simulink model "pendulum_openloop"  (R2026a)
settings: Solver=VariableStepAuto
values from neighbouring files (symbols this model uses):
  p = [ ... (first row only)    [init_pendulum.m]
  q0 = [ ... (first row only)    [init_pendulum.m]
  qd0 = [ ... (first row only)    [init_pendulum.m]
  u0 = [ ... (first row only)    [init_pendulum.m]
settings Model: Creator=vb  LastModifiedBy=vb

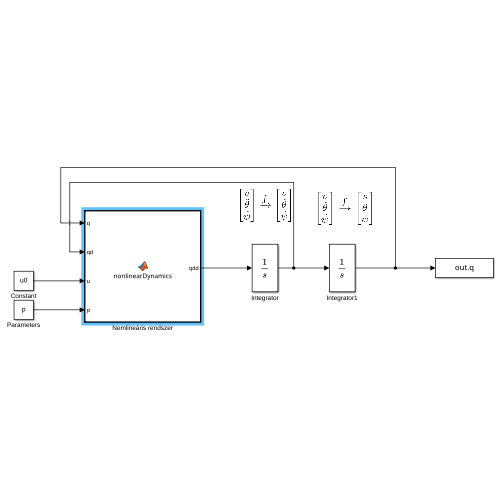
[thumbnail: Simulink's stored preview of the top-level diagram]
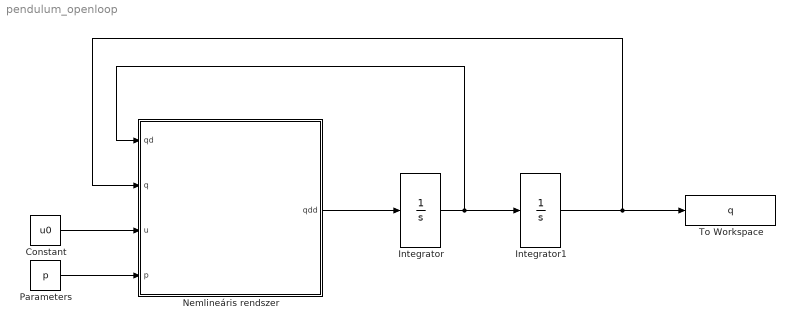
== system pendulum_openloop ==
  Constant : Constant  Value=u0
  Integrator : Integrator  InitialCondition=qd0
  Integrator1 : Integrator  InitialCondition=q0
  Nemlineáris rendszer : MATLAB Function  TreatAsAtomicUnit=on
  Parameters : Constant  Value=p
  To Workspace : ToWorkspace  VariableName=q  SaveFormat=Timeseries  SampleTime=-1
  wires:
  Nemlineáris rendszer/1(qdd) -> Integrator/1
  Integrator/1 -> Nemlineáris rendszer/1(qd), Integrator1/1
  Integrator1/1 -> To Workspace/1, Nemlineáris rendszer/2(q)
  Constant/1 -> Nemlineáris rendszer/3(u)
  Parameters/1 -> Nemlineáris rendszer/4(p)

== matlab function pendulum_openloop/Nemlineáris rendszer ==
  data: qd input; q input; u input; qdd output; p input
function qdd = nonlinearDynamics(qd, q, u, p)

% q  = [s, theta, psi]
% qd = [v, thetaDot, psiDot]
% u  = [tauCommon, tauDifferential]

%% Alap fizikai paraméterek

mb  = p(1);
mw  = p(2);
r   = p(3);
b   = p(4);
l   = p(5);

Ix  = p(6);
Iy  = p(7);
Iz  = p(8);

Ja  = p(9);
Jzw = p(10);

g   = p(11);

%% Súrlódási / veszteségi paraméterek

cMotor   = p(12);   % motor+csapágy viszkózus súrlódás [Nms/rad]
tauMotor = p(13);   % motor+csapágy Coulomb súrlódás [Nm]

cRoll    = p(14);   % gördülési viszkózus ellenállás [Ns/m]
FRoll    = p(15);   % gördülési Coulomb jellegű ellenállás [N]

cAir     = p(16);   % légellenállási együttható

vEps     = p(17);   % simítási sebesség [m/s]
omegaEps = p(18);   % simítási szögsebesség [rad/s]


%% Állapotok

v        = qd(1);
theta    = q(2);
thetaDot = qd(2);
psiDot   = qd(3);


%% Összevont tehetetlenségek

A = mb + 2*mw + 2*Ja/r^2;

C = Iy + mb*l^2;

D = Ix*sin(theta)^2 ...
  + Iz*cos(theta)^2 ...
  + mb*l^2*sin(theta)^2 ...
  + mw*b^2/2 ...
  + Ja*b^2/(2*r^2) ...
  + 2*Jzw;

Dp = 2*sin(theta)*cos(theta) ...
   * (Ix - Iz + mb*l^2);


%% Tömegmátrix

M = [
    A,                  mb*l*cos(theta), 0;
    mb*l*cos(theta),    C,               0;
    0,                  0,               D
];


%% Nemlineáris konzervatív tagok

h = [
    -mb*l*sin(theta)*thetaDot^2;
    -0.5*Dp*psiDot^2 - mb*g*l*sin(theta);
    Dp*thetaDot*psiDot
];


%% Bemeneti mátrix

B = [
     2/r, 0;
    -2,   0;
     0,   b/r
];


%% ------------------------------------------------------------
% Keréksebességek
% ------------------------------------------------------------

vL = v - b/2*psiDot;
vR = v + b/2*psiDot;

omegaL = vL/r;
omegaR = vR/r;


%% ------------------------------------------------------------
% Motor / csapágy relatív szögsebességek
% ------------------------------------------------------------

alphaDotL = omegaL - thetaDot;
alphaDotR = omegaR - thetaDot;


%% ------------------------------------------------------------
% Motor + csapágy súrlódási nyomaték
% ------------------------------------------------------------

tauFricL = cMotor*alphaDotL ...
         + tauMotor*tanh(alphaDotL/omegaEps);

tauFricR = cMotor*alphaDotR ...
         + tauMotor*tanh(alphaDotR/omegaEps);


% közös / különbségi komponensek

tauFricCommon = (tauFricL + tauFricR)/2;
tauFricDiff   = (tauFricR - tauFricL)/2;

uFric = [
    tauFricCommon;
    tauFricDiff
];

QmotorFric = -B*uFric;


%% ------------------------------------------------------------
% Gördülési ellenállás
% ------------------------------------------------------------

FrollL = cRoll*vL ...
       + FRoll*tanh(vL/vEps);

FrollR = cRoll*vR ...
       + FRoll*tanh(vR/vEps);

Qroll = [
    -(FrollL + FrollR);
     0;
    -b/2*(FrollR - FrollL)
];


%% ------------------------------------------------------------
% Légellenállás
% ------------------------------------------------------------

Fair = cAir*v*abs(v);

Qair = [
    -Fair;
     0;
     0
];


%% ------------------------------------------------------------
% Teljes disszipatív általánosított erő
% ------------------------------------------------------------

Qfriction = QmotorFric + Qroll + Qair;


%% ------------------------------------------------------------
% Mozgásegyenlet
% ------------------------------------------------------------

qdd = M \ (B*u + Qfriction - h);

end
